simulink model "scheme2"  (R2026b)
settings: Solver=VariableStepAuto
settings Model: Creator=vladi  LastModifiedBy=misha

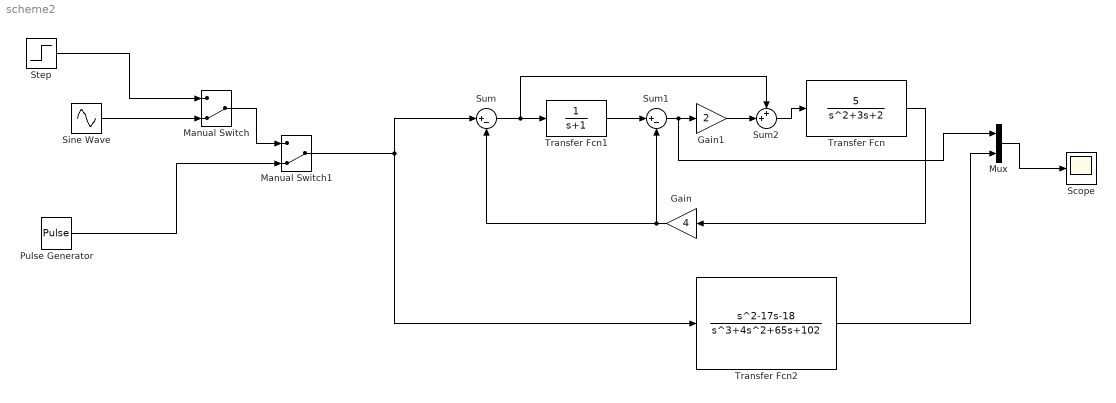
== system scheme2 ==
  Gain : Gain  Gain=4
  Gain1 : Gain  Gain=2
  Manual Switch : ManualSwitch  CurrentSetting=0
  Manual Switch1 : ManualSwitch  CurrentSetting=0
  Mux : Mux  Inputs=2
  Pulse Generator : DiscretePulseGenerator  PulseType=Time based  Amplitude=100  Period=20  PulseWidth=0.05  PhaseDelay=1
  Scope : Scope
      settings: ActiveDisplayYMinimum=-0.490879646475056  ActiveDisplayYMaximum=0.080477790359126347
  Sine Wave : Sin  SampleTime=0
  Step : Step  SampleTime=0
  Sum : Sum  Inputs=|+-
  Sum1 : Sum  Inputs=|+-
  Sum2 : Sum  Inputs=++|
  Transfer Fcn : TransferFcn  Numerator=[5]  Denominator=[1 3 2]
  Transfer Fcn1 : TransferFcn  Denominator=[1 1]
  Transfer Fcn2 : TransferFcn  Numerator=[1 -17 -18]  Denominator=[1 4 65 102]
  wires:
  Sum/1 -> Sum2/1, Transfer Fcn1/1
  Transfer Fcn1/1 -> Sum1/1
  Gain1/1 -> Sum2/2
  Sum2/1 -> Transfer Fcn/1
  Transfer Fcn/1 -> Gain/1
  Gain/1 -> Sum1/2, Sum/2
  Sum1/1 -> Mux/1, Gain1/1
  Transfer Fcn2/1 -> Mux/2
  Mux/1 -> Scope/1
  Step/1 -> Manual Switch/1
  Sine Wave/1 -> Manual Switch/2
  Pulse Generator/1 -> Manual Switch1/2
  Manual Switch/1 -> Manual Switch1/1
  Manual Switch1/1 -> Sum/1, Transfer Fcn2/1
